simulink model "finalmodel2"  (R2024b)
settings: Solver=ode4  StartTime=0.0  StopTime=110.0  FixedStep=SampleTime  MaxStep=1e-3  RelTol=1e-4  AbsTol=1e-3
values from neighbouring files (symbols this model uses):
  Cf = 0.00911825194797    [finalmodel2.mat]    (also in finalmodel3.mat)
  D = 6191.85011148    [finalmodel2.mat]    (also in finalmodel3.mat)
  J = 773.981263935    [finalmodel2.mat]    (also in finalmodel3.mat)
  k10 = 1    [finalmodel2.mat]    (also in finalmodel3.mat)
  k11 = 25    [finalmodel2.mat]    (also in finalmodel3.mat)
  k12 = 1    [finalmodel2.mat]    (also in finalmodel3.mat)
  k13 = 120    [finalmodel2.mat]    (also in finalmodel3.mat)
  k14 = 1    [finalmodel2.mat]    (also in finalmodel3.mat)
  k2 = 9.4    [finalmodel2.mat]    (also in finalmodel3.mat)
  k3 = 1    [finalmodel2.mat]    (also in finalmodel3.mat)
  k4 = 25    [finalmodel2.mat]    (also in finalmodel3.mat)
  k5 = 1    [finalmodel2.mat]    (also in finalmodel3.mat)
  k6 = 120    [finalmodel2.mat]    (also in finalmodel3.mat)
  k7 = 1    [finalmodel2.mat]    (also in finalmodel3.mat)
  k9 = 9.4    [finalmodel2.mat]    (also in finalmodel3.mat)
  Kip_vsg = 0.00606060606061    [finalmodel2.mat]    (also in finalmodel3.mat)
  Kq_vsg = 1.48453923805e-06    [finalmodel2.mat]    (also in finalmodel3.mat)
  Kvi_vsg = 899.93539556    [finalmodel2.mat]    (also in finalmodel3.mat)
  Kvp_vsg = 5.72916666667    [finalmodel2.mat]    (also in finalmodel3.mat)
  L1 = 1.15749049521e-05    [finalmodel2.mat]    (also in finalmodel3.mat)
  Ls = 1.92915082536e-06    [finalmodel2.mat]    (also in finalmodel3.mat)
  Pset = 8281000    [finalmodel2.mat]    (also in finalmodel3.mat = 8280000)
  R1 = 0.000290909090909    [finalmodel2.mat]    (also in finalmodel3.mat)
  SampleTime = 5e-05    [finalmodel2.mat]    (also in finalmodel3.mat)
  Us = 326.598632371    [finalmodel2.mat]    (also in finalmodel3.mat)
  Vdclink = 800    [finalmodel2.mat]    (also in finalmodel3.mat)
  wn = 376.991118431    [finalmodel2.mat]    (also in finalmodel3.mat)
undefined symbols (not defined in the file or in its folder): sigbuilder_block
libraries: spsThreePhaseVIMeasurementLib x15, spsLoadFlowBusLib x9, spsThreePhasePISectionLineLib x6, spsThreePhaseTransformerTwoWindingsLib x4, spsThreePhaseParallelRLCLoadLib x4, spsabctodq0Lib x4, spsThreePhaseSeriesRLCBranchLib x3, spsSynchronousMachinepuStandardLib x2, spsExcitationSystemLib x2, spsMultiBandPowerSystemStabilizerLib x2, spsSteamTurbineandGovernorLib x2, spsGroundLib x2
(part 1 of 3)
settings Model: SimulationMode=accelerator  Creator=jp536285  LastModifiedBy=Raju
settings SolverCC: AutoScaleAbsTol=off  InitialStep=1e-5  ZeroCrossControl=DisableAll  AlgebraicLoopSolver=TrustRegion  AutoInsertRateTranBlk=on
settings DataIOCC: MaxDataPoints=100000
settings OptimizationCC: LifeSpan=inf
settings DebuggingCC: UnderspecifiedInitializationDetection=Classic  MergeDetectMultiDrivingBlocksExec=none  MultiTaskRateTransMsg=warning  IntegerOverflowMsg=none  StateNameClashWarn=warning  SFUnexpectedBacktrackingDiag=warning  SFNoUnconditionalDefaultTransitionDiag=warning  ArithmeticOperatorsInVariantConditions=warning
settings HardwareCC: ProdBitPerPointer=32  ProdBitPerSizeT=32  ProdBitPerPtrDiffT=32  ProdLargestAtomicFloat=None  ProdIntDivRoundTo=Undefined  ProdEndianess=Unspecified  ProdWordSize=32  ProdHWDeviceType=32-bit Generic
settings ModelReferenceCC: EnableRefExpFcnMdlSchedulingChecks=on  PropagateSignalLabelsOutOfModel=off
settings SFSimCC: SimUseLocalCustomCode=off  CustomCodeUndefinedFunction=UseInterfaceOnly
settings RTWCC: RTWUseLocalCustomCode=off  GPUComputeCapability=3.5
settings CodeAppCC: StateflowObjectComments=on
settings GRTTargetCC: TargetLangStandard=C89/C90 (ANSI)
settings ConfigComp: CovMetricSettings=dw  CovSaveCumulativeToWorkspaceVar=on  CovSaveSingleToWorkspaceVar=on  CovExternalEMLEnable=off
settings SimscapeCC: SimscapeNormalizeSystem=off

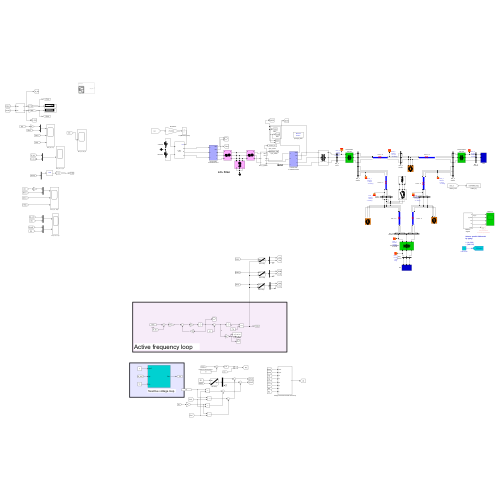
[thumbnail: Simulink's stored preview of the top-level diagram]
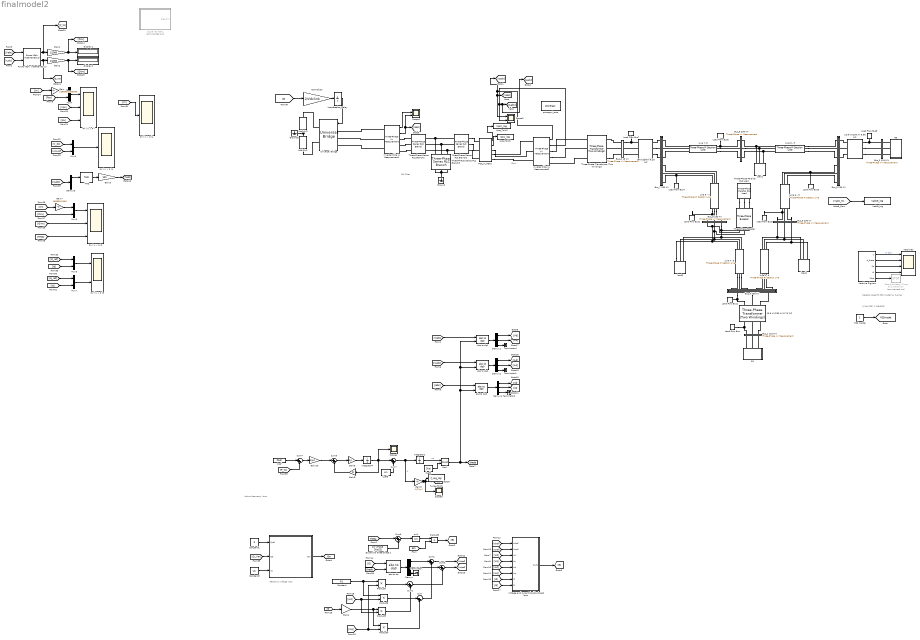
== system finalmodel2 ==
  note: Select a specific PSS model
      | by typing:
  note: 0  (No PSS)
      | 1  (MB-PSS)
  note: Grid
  note: LCL Filter
  note: Reactive voltage loop
  note: Active frequency loop
  " " : Subsystem
  " Line 4 - 6" : spsThreePhasePISectionLineLib/Three-Phase PI Section Line  LConnTagsString=a|b|c  RConnTagsString=A|B|C  Length=100  Frequency=60  Resistances=[ 0.08993 0.224825]  Inductances="[ 1.29e-3  3.22e-3]"  Capacitances="[ 9.5e-9  6.5e-9 ]"  mask(Three-Phase PI Section Line){}
      mask Display:
      | % This is a new mask on top of the base mask.
      | % Use "View base mask" link below to see the base mask.
      | patch([0.0 0.0 1 1 0.0 0.0 ],[0.4 0.7 0.7 0.4 0.4 0.7],[0 0 1]);
      | patch([0.4 0.4 0.42 0.42],[0.4 0.75 0.75 0.4],[1 0 0]);
      | patch([0.38 0.38 0.57 0.57],[0.7 0.75 0.75 0.7],[1 0 0]);
      | patch([0.53 0.53 0.55 0.55],[0.4 0.75 0.75 0.4],[1 0 0]);
  " Line 6 - 9" : spsThreePhasePISectionLineLib/Three-Phase PI Section Line  LConnTagsString=a|b|c  RConnTagsString=A|B|C  Length=100  Frequency=60  Resistances=[ 0.20631 0.5157]  Inductances="[ 2.38e-3  6.09e-3]"  Capacitances=[17.95e-9 10.55e-9]  mask(Three-Phase PI Section Line){}
      mask Display:
      | % This is a new mask on top of the base mask.
      | % Use "View base mask" link below to see the base mask.
      | patch([0.0 0.0 1 1 0.0 0.0 ],[0.4 0.7 0.7 0.4 0.4 0.7],[0 0 1]);
      | patch([0.4 0.4 0.42 0.42],[0.4 0.75 0.75 0.4],[1 0 0]);
      | patch([0.38 0.38 0.57 0.57],[0.7 0.75 0.75 0.7],[1 0 0]);
      | patch([0.53 0.53 0.55 0.55],[0.4 0.75 0.75 0.4],[1 0 0]);
  13.8 KV/230 KV 5.86 %Z : spsThreePhaseTransformerTwoWindingsLib/Three-Phase Transformer (Two Windings)  Winding1Connection=Yg  Winding2Connection=Yg  CoreType=Three single-phase transformers  SetSaturation=off  Hysteresis=off  DataFile='hysteresis'  SetInitialFlux=off  Measurements=None  UNITS=pu  NominalPower=[ 100e6 , 60 ]  Winding1=[ 13.8e3 , 1e-6 , 0 ]  Winding2=[ 230e3 , 1e-6, 0.0586 ]  Rm=500  Lm=500  L0=0.5  Saturation=[ 0,0 ; 0.0024,1.2 ; 1.0,1.52 ]  InitialFluxes=[ 0.8 , -0.8 , 0.7 ]  BreakLoop=off  DiscreteSolver=Trapezoidal iterative  DataType=off  TransfoNumber=1
  "16.5 KV/230 KV 5.76 %Z     " : spsThreePhaseTransformerTwoWindingsLib/Three-Phase Transformer (Two Windings)  Winding1Connection=Yg  Winding2Connection=Yg  CoreType=Three single-phase transformers  SetSaturation=off  Hysteresis=off  DataFile='hysteresis'  SetInitialFlux=off  Measurements=None  UNITS=pu  NominalPower=[ 100e6 , 60 ]  Winding1=[ 16.5e3 , 1e-6, 0 ]  Winding2=[ 230e3 ,1e-6, 0.0576 ]  Rm=500  Lm=500  L0=0.5  Saturation=[ 0,0 ; 0.0024,1.2 ; 1.0,1.52 ]  InitialFluxes=[ 0.8 , -0.8 , 0.7 ]  BreakLoop=off  DiscreteSolver=Trapezoidal iterative  DataType=off  TransfoNumber=1
  18KV/230KV 6.25 %Z : spsThreePhaseTransformerTwoWindingsLib/Three-Phase Transformer (Two Windings)  Winding1Connection=Yg  Winding2Connection=Yg  CoreType=Three single-phase transformers  SetSaturation=off  Hysteresis=off  DataFile='hysteresis'  SetInitialFlux=off  Measurements=None  UNITS=pu  NominalPower=[ 100e6 , 60 ]  Winding1=[ 18e3 , 1e-6 , 0]  Winding2=[ 230e3 , 1e-6, 0.0625 ]  Rm=500  Lm=500  L0=0.5  Saturation=[ 0,0 ; 0.0024,1.2 ; 1.0,1.52 ]  InitialFluxes=[ 0.8 , -0.8 , 0.7 ]  BreakLoop=off  DiscreteSolver=Trapezoidal iterative  DataType=off  TransfoNumber=1
  Bus_1 16.5 KV : spsThreePhaseVIMeasurementLib/Three-Phase V-I Measurement  VoltageMeasurement=phase-to-ground  SetLabelV=on  LabelV=Vabc_1  Vpu=on  VpuLL=off  CurrentMeasurement=yes  SetLabelI=on  LabelI=Iabc_1  Ipu=on  Pbase=100e6  Vbase=16.5e3  OutputType=Complex  PhasorSimulation=off  PSBequivalent=0
  Bus_2 18 KV : spsThreePhaseVIMeasurementLib/Three-Phase V-I Measurement  VoltageMeasurement=phase-to-ground  SetLabelV=on  LabelV=Vabc_2  Vpu=on  VpuLL=off  CurrentMeasurement=yes  SetLabelI=on  LabelI=Iabc_2  Ipu=on  Pbase=100e6  Vbase=18e3  OutputType=Complex  PhasorSimulation=off  PSBequivalent=0
  Bus_3 13.8 KV : spsThreePhaseVIMeasurementLib/Three-Phase V-I Measurement  VoltageMeasurement=phase-to-ground  SetLabelV=on  LabelV=Vabc_3  Vpu=on  VpuLL=off  CurrentMeasurement=yes  SetLabelI=on  LabelI=Iabc_3  Ipu=on  Pbase=100e6  Vbase=13.8e3  OutputType=Complex  PhasorSimulation=off  PSBequivalent=0
  Bus_4 230 KV : Subsystem
  Bus_5 230 KV : spsThreePhaseVIMeasurementLib/Three-Phase V-I Measurement  VoltageMeasurement=phase-to-ground  SetLabelV=on  LabelV=Vabc_5  Vpu=on  VpuLL=off  CurrentMeasurement=yes  SetLabelI=on  LabelI=Iabc_5  Ipu=on  Pbase=100e6  Vbase=230e3  OutputType=Complex  PhasorSimulation=off  PSBequivalent=0
  Bus_6 230 KV : spsThreePhaseVIMeasurementLib/Three-Phase V-I Measurement  VoltageMeasurement=phase-to-phase  SetLabelV=on  LabelV=Vabc_6  Vpu=off  VpuLL=on  CurrentMeasurement=yes  SetLabelI=on  LabelI=Iabc_6  Ipu=on  Pbase=100e6  Vbase=230e3  OutputType=Complex  PhasorSimulation=off  PSBequivalent=0
  Bus_7 230 KV : Subsystem
  Bus_8 230 KV : spsThreePhaseVIMeasurementLib/Three-Phase V-I Measurement  VoltageMeasurement=phase-to-phase  SetLabelV=on  LabelV=Vabc_8  Vpu=off  VpuLL=on  CurrentMeasurement=yes  SetLabelI=on  LabelI=Iabc_8  Ipu=on  Pbase=100e6  Vbase=230e3  OutputType=Complex  PhasorSimulation=off  PSBequivalent=0
  Bus_9 230 KV : Subsystem
  Constant : Constant  Value=R1
  Constant1 : Constant  Value=0
  Constant2 : Constant  Value=Us
  Demux{,1..4} (5 alike) : Demux  Outputs=3
      Demux1 settings: DisplayOption=none
      Demux2 settings: DisplayOption=none
      Demux4 settings: DisplayOption=none
  Display1 : Display
      settings: SampleTime=SampleTime
  Display2 : Display
      settings: SampleTime=SampleTime
  Expand to three-phase 1 : Constant  Value=[0 -2*pi/3 2*pi/3]
  G1 : Subsystem
  G3 : Subsystem
  Gain : Gain  Gain=108830/1000000  SampleTime=SampleTime
  Gain1 : Gain  Gain=1/1000  SampleTime=SampleTime
  Gain10 : Gain  Gain=1/wn
  Gain2 : Gain  Gain=1/1000  SampleTime=SampleTime
  Gain3 : Gain  Gain=100  SampleTime=SampleTime
  Gain4 : Gain  Gain=L1*2*pi
  Gain5 : Gain  Gain=1/J
  Gain7 : Gain  Gain=108830/1000  SampleTime=SampleTime
  Gain8 : Gain  Gain=D
  Gain9 : Gain  Gain=1/(2*pi)
  "Ground " : spsGroundLib/Ground  LConnTagsString=a
  Ground3 : spsGroundLib/Ground  LConnTagsString=a
  Integrator1 : Integrator
  Integrator4 : Integrator
  Inverter Side V-I Measurement1 : spsThreePhaseVIMeasurementLib/Three-Phase V-I Measurement  VoltageMeasurement=phase-to-phase  SetLabelV=off  LabelV=Vabc  Vpu=off  VpuLL=off  CurrentMeasurement=yes  SetLabelI=off  LabelI=Iabc  Ipu=off  Pbase=100e6  Vbase=500e3  OutputType=Complex  PhasorSimulation=off  PSBequivalent=0
  Inverter Side V-I Measurement2 : spsThreePhaseVIMeasurementLib/Three-Phase V-I Measurement  VoltageMeasurement=phase-to-ground  SetLabelV=off  LabelV=Vabc  Vpu=off  VpuLL=off  CurrentMeasurement=yes  SetLabelI=off  LabelI=Iabc  Ipu=off  Pbase=100e6  Vbase=500e3  OutputType=Complex  PhasorSimulation=off  PSBequivalent=0
  Ipcc_ToWS : ToWorkspace  VariableName=Ipcc_log  SaveFormat=Timeseries  SampleTime=SampleTime
  "Line 4 - 5 " : spsThreePhasePISectionLineLib/Three-Phase PI Section Line  LConnTagsString=a|b|c  RConnTagsString=A|B|C  Length=100  Frequency=60  Resistances=[ 0.0529 0.13225]  Inductances="[ 1.192e-3  2.38e-3]"  Capacitances="[ 9.5e-9  6.5e-9 ]"  mask(Three-Phase PI Section Line){}
      mask Display:
      | % This is a new mask on top of the base mask.
      | % Use "View base mask" link below to see the base mask.
      | patch([0.0 0.0 1 1 0.0 0.0 ],[0.4 0.7 0.7 0.4 0.4 0.7],[0 0 1]);
      | patch([0.4 0.4 0.42 0.42],[0.4 0.75 0.75 0.4],[1 0 0]);
      | patch([0.38 0.38 0.57 0.57],[0.7 0.75 0.75 0.7],[1 0 0]);
      | patch([0.53 0.53 0.55 0.55],[0.4 0.75 0.75 0.4],[1 0 0]);
  "Line 5 - 7 " : spsThreePhasePISectionLineLib/Three-Phase PI Section Line  LConnTagsString=a|b|c  RConnTagsString=A|B|C  Length=100  Frequency=60  Resistances=[ 0.16928 0.4232]  Inductances="[ 2.259e-3  5.64e-3]"  Capacitances=[15.34e-9 9.025e-9]  mask(Three-Phase PI Section Line){}
      mask Display:
      | % This is a new mask on top of the base mask.
      | % Use "View base mask" link below to see the base mask.
      | patch([0.0 0.0 1 1 0.0 0.0 ],[0.4 0.7 0.7 0.4 0.4 0.7],[0 0 1]);
      | patch([0.4 0.4 0.42 0.42],[0.4 0.75 0.75 0.4],[1 0 0]);
      | patch([0.38 0.38 0.57 0.57],[0.7 0.75 0.75 0.7],[1 0 0]);
      | patch([0.53 0.53 0.55 0.55],[0.4 0.75 0.75 0.4],[1 0 0]);
  Line 7- 8 : spsThreePhasePISectionLineLib/Three-Phase PI Section Line  LConnTagsString=a|b|c  RConnTagsString=A|B|C  Length=100  Frequency=60  Resistances=[0.044965 0.11241]  Inductances="[ 1.01e-3  2.02e-3]"  Capacitances="[ 12.5e-9  6.5e-9 ]"  mask(Three-Phase PI Section Line){}
      mask Display:
      | % This is a new mask on top of the base mask.
      | % Use "View base mask" link below to see the base mask.
      | patch([0.0 0.0 1 1 0.0 0.0 ],[0.4 0.7 0.7 0.4 0.4 0.7],[0 0 1]);
      | patch([0.4 0.4 0.42 0.42],[0.4 0.75 0.75 0.4],[1 0 0]);
      | patch([0.38 0.38 0.57 0.57],[0.7 0.75 0.75 0.7],[1 0 0]);
      | patch([0.53 0.53 0.55 0.55],[0.4 0.75 0.75 0.4],[1 0 0]);
  Line 8 - 9 : spsThreePhasePISectionLineLib/Three-Phase PI Section Line  LConnTagsString=a|b|c  RConnTagsString=A|B|C  Length=100  Frequency=60  Resistances=[ 0.062951 0.15737]  Inductances="[ 1.414e-3  3.53e-3]"  Capacitances=[10.47e-9 6.15e-9]  mask(Three-Phase PI Section Line){}
      mask Display:
      | % This is a new mask on top of the base mask.
      | % Use "View base mask" link below to see the base mask.
      | patch([0.0 0.0 1 1 0.0 0.0 ],[0.4 0.7 0.7 0.4 0.4 0.7],[0 0 1]);
      | patch([0.4 0.4 0.42 0.42],[0.4 0.75 0.75 0.4],[1 0 0]);
      | patch([0.38 0.38 0.57 0.57],[0.7 0.75 0.75 0.7],[1 0 0]);
      | patch([0.53 0.53 0.55 0.55],[0.4 0.75 0.75 0.4],[1 0 0]);
  Load Flow Bus : spsLoadFlowBusLib/Load Flow Bus  LConnTagsString=a  Phases=single  Connectors=on one side  ID=BUS_1  Vbase=16.5e3  Vref=1.04  Vangle=0  VLF=1.04  VLFb=1  VLFc=1  angleLF=0  angleLFb=0  angleLFc=0
      settings: AttributesFormatString=%<ID>\n%<Vbase>V\n%<VLF>pu\n%<angleLF>deg.
  Load Flow Bus1 : spsLoadFlowBusLib/Load Flow Bus  LConnTagsString=a  Phases=single  Connectors=on one side  ID=BUS_4  Vbase=230e3  Vref=1  Vangle=0  VLF=1.029  VLFb=1  VLFc=1  angleLF=-7.275  angleLFb=0  angleLFc=0
      settings: AttributesFormatString=%<ID>\n%<Vbase>V\n%<VLF>pu\n%<angleLF>deg.
  Load Flow Bus2 : spsLoadFlowBusLib/Load Flow Bus  LConnTagsString=a  Phases=single  Connectors=on one side  ID=BUS_5  Vbase=230e3  Vref=1  Vangle=0  VLF=1.002  VLFb=1  VLFc=1  angleLF=-13.97  angleLFb=0  angleLFc=0
      settings: AttributesFormatString=%<ID>\n%<Vbase>V\n%<VLF>pu\n%<angleLF>deg.
  Load Flow Bus3 : spsLoadFlowBusLib/Load Flow Bus  LConnTagsString=a  Phases=single  Connectors=on one side  ID=BUS_6  Vbase=230e3  Vref=1  Vangle=0  VLF=1.017  VLFb=1  VLFc=1  angleLF=-11.82  angleLFb=0  angleLFc=0
      settings: AttributesFormatString=%<ID>\n%<Vbase>V\n%<VLF>pu\n%<angleLF>deg.
  Load Flow Bus4 : spsLoadFlowBusLib/Load Flow Bus  LConnTagsString=a  Phases=single  Connectors=on one side  ID=BUS_7  Vbase=230e3  Vref=1  Vangle=0  VLF=1.025  VLFb=1  VLFc=1  angleLF=-15.86  angleLFb=0  angleLFc=0
      settings: AttributesFormatString=%<ID>\n%<Vbase>V\n%<VLF>pu\n%<angleLF>deg.
  Load Flow Bus5 : spsLoadFlowBusLib/Load Flow Bus  LConnTagsString=a  Phases=single  Connectors=on one side  ID=BUS_9  Vbase=230e3  Vref=1  Vangle=0  VLF=1.031  VLFb=1  VLFc=1  angleLF=-11.92  angleLFb=0  angleLFc=0
      settings: AttributesFormatString=%<ID>\n%<Vbase>V\n%<VLF>pu\n%<angleLF>deg.
  Load Flow Bus6 : spsLoadFlowBusLib/Load Flow Bus  LConnTagsString=a  Phases=single  Connectors=on one side  ID=BUS_8  Vbase=230e3  Vref=1  Vangle=0  VLF=1.017  VLFb=1  VLFc=1  angleLF=-16.48  angleLFb=0  angleLFc=0
      settings: AttributesFormatString=%<ID>\n%<Vbase>V\n%<VLF>pu\n%<angleLF>deg.
  Load Flow Bus7 : spsLoadFlowBusLib/Load Flow Bus  LConnTagsString=a  Phases=single  Connectors=on one side  ID=BUS_2  Vbase=18e3  Vref=1.025  Vangle=0  VLF=1.025  VLFb=1  VLFc=1  angleLF=-15.88  angleLFb=0  angleLFc=0
      settings: AttributesFormatString=%<ID>\n%<Vbase>V\n%<VLF>pu\n%<angleLF>deg.
  Load Flow Bus8 : spsLoadFlowBusLib/Load Flow Bus  LConnTagsString=a  Phases=single  Connectors=on one side  ID=BUS_3  Vbase=13.8e3  Vref=1.025  Vangle=0  VLF=1.025  VLFb=1  VLFc=1  angleLF=-9.229  angleLFb=0  angleLFc=0
      settings: AttributesFormatString=%<ID>\n%<Vbase>V\n%<VLF>pu\n%<angleLF>deg.
  LoopBreaker_Delay : UnitDelay  SampleTime=SampleTime  HasFrameUpgradeWarning=on
  Machine Signals : Subsystem
  Machines : Scope  NumInputPorts=4
  Mod : Math  Operator=mod  SignedPower=on
  Mux{3..7} (5 alike) : Mux  Inputs=2
  Normalizer : Gain  Gain=2/Vdclink
  PCC_VI_Meas : spsThreePhaseVIMeasurementLib/Three-Phase V-I Measurement  VoltageMeasurement=phase-to-ground  SetLabelV=off  LabelV=Vabc  Vpu=off  VpuLL=off  CurrentMeasurement=yes  SetLabelI=off  LabelI=Iabc  Ipu=off  Pbase=100e6  Vbase=500e3  OutputType=Complex  PhasorSimulation=off  PSBequivalent=0
  PSS model : Constant  SampleTime=SampleTime
  "PV ( V, I, P )" : Scope  NumInputPorts=3
  "PV ( V, I, P )1" : Scope
  "PV ( V, I, P )2" : Scope  NumInputPorts=3
  "PV ( V, I, P )3" : Scope  NumInputPorts=2
  "PV ( V, I, P )4" : Scope
  "Power (3ph, Instantaneous)" : spsPower3phInstantaneousLib/Power (3ph, Instantaneous)
  Pref : Constant  Value=Pset
  Product{3..7} (5 alike) : Product
  Scope1 : Scope  NumInputPorts=2
  Scope2 : Scope  NumInputPorts=2
  Scope3 : Scope
  Scope4 : Scope
  Signal Builder2 : Subsystem  Tag=STV Subsys  Commented=on  LoadFcn=sigbuilder_block('load');  StartFcn=sigbuilder_block('start');  StopFcn=sigbuilder_block('stop');  ClipboardFcn=sigbuilder_block('clipboard');  mask(Sigbuilder block){tuvar=[0:10]}
      mask help: Simulink:masks:SigbuilderBlock_MD
      mask init:
      | if ~strcmp(get_param(bdroot(gcbh),'SimulationStatus'),'stopped') tuvar = sigbuilder_block('maskInit'); end
      settings: CopyFcn=sigbuilder_block('copy');  DeleteFcn=sigbuilder_block('delete');  ModelCloseFcn=sigbuilder_block('modelClose');  PreSaveFcn=sigbuilder_block('preSave');  PauseFcn=sigbuilder_block('pause');  ContinueFcn=sigbuilder_block('continue');  NameChangeFcn=sigbuilder_block('namechange');  OpenFcn=sigbuilder_block('open',[220.2 153.6 550.8 361.2 ]);  CloseFcn=sigbuilder_block('close');
      mask Display: plot(0, 0, 100, 100,[2, 2, 32, 32, 2], [68, 8, 8, 68, 68],[32, 2], [38, 38], [32, 19, 2],[53, 60, 44], [32, 17, 17, 2],[16, 16, 31, 31]);txt = getActiveGroup(gcbh);text(2, 100, txt,'verticalAlignment', 'top');
  Stop simulation if loss of synchronism : Stop  Commented=on
  Sum : Sum  Inputs=|-+
  Sum{1..2,6..7} (4 alike) : Sum  Inputs=|++
  Sum3 : Sum  Inputs=|+-
  Sum4 : Sum  Inputs=|+-
  Sum5 : Sum  Inputs=|+-
  THD : spsTHDLib/THD  Freq=50  Ts=SampleTime
      link override In: SampleTime=SampleTime
      link override Mean: Ts=SampleTime
      link override Mean/In: SampleTime=SampleTime
      link override Mean/Mean: SampleTime=SampleTime
      link override Mean/Model/Digital  Clock: SampleTime=SampleTime
      link override Mean/Model/Discrete Variable Time Delay: Ts=SampleTime
      link override Mean/Model/Discrete Variable Time Delay/D: SampleTime=SampleTime
      link override Mean/Model/Discrete Variable Time Delay/In: SampleTime=SampleTime
      link override Mean/Model/Discrete Variable Time Delay/Out: SampleTime=SampleTime
      link override Mean/Model/Integ4: SampleTime=SampleTime
      link override Mean/Model/K1: SampleTime=SampleTime
      link override Mean/Model/K2: SampleTime=SampleTime
      link override Mean/Model/Relational Operator: SampleTime=SampleTime
      link override Mean/Model/Unit Delay: SampleTime=SampleTime
      link override Mean/Model/Unit Delay1: SampleTime=SampleTime
      link override RMS1: Ts=SampleTime
      link override RMS1/In: SampleTime=SampleTime
      link override RMS1/RMS: SampleTime=SampleTime
      link override RMS1/RMS /Fourier1: Ts=SampleTime
      link override RMS1/RMS /Fourier1/In: SampleTime=SampleTime
      link override RMS1/RMS /Fourier1/Mag: SampleTime=SampleTime
      link override RMS1/RMS /Fourier1/Mean: Ts=SampleTime
      link override RMS1/RMS /Fourier1/Mean value1: Ts=SampleTime
      link override RMS1/RMS /Fourier1/Mean value1/In: SampleTime=SampleTime
      link override RMS1/RMS /Fourier1/Mean value1/Mean: SampleTime=SampleTime
      link override RMS1/RMS /Fourier1/Mean value1/Model/Digital  Clock: SampleTime=SampleTime
      link override RMS1/RMS /Fourier1/Mean value1/Model/Discrete Variable Time Delay: Ts=SampleTime
      link override RMS1/RMS /Fourier1/Mean value1/Model/Discrete Variable Time Delay/D: SampleTime=SampleTime
      link override RMS1/RMS /Fourier1/Mean value1/Model/Discrete Variable Time Delay/In: SampleTime=SampleTime
      link override RMS1/RMS /Fourier1/Mean value1/Model/Discrete Variable Time Delay/Out: SampleTime=SampleTime
      link override RMS1/RMS /Fourier1/Mean value1/Model/Integ4: SampleTime=SampleTime
      link override RMS1/RMS /Fourier1/Mean value1/Model/K1: SampleTime=SampleTime
      link override RMS1/RMS /Fourier1/Mean value1/Model/K2: SampleTime=SampleTime
      link override RMS1/RMS /Fourier1/Mean value1/Model/Relational Operator: SampleTime=SampleTime
      link override RMS1/RMS /Fourier1/Mean value1/Model/Unit Delay: SampleTime=SampleTime
      link override RMS1/RMS /Fourier1/Mean value1/Model/Unit Delay1: SampleTime=SampleTime
      link override RMS1/RMS /Fourier1/Mean/In: SampleTime=SampleTime
      link override RMS1/RMS /Fourier1/Mean/Mean: SampleTime=SampleTime
      link override RMS1/RMS /Fourier1/Mean/Model/Digital  Clock: SampleTime=SampleTime
      link override RMS1/RMS /Fourier1/Mean/Model/Discrete Variable Time Delay: Ts=SampleTime
      link override RMS1/RMS /Fourier1/Mean/Model/Discrete Variable Time Delay/D: SampleTime=SampleTime
      link override RMS1/RMS /Fourier1/Mean/Model/Discrete Variable Time Delay/In: SampleTime=SampleTime
      link override RMS1/RMS /Fourier1/Mean/Model/Discrete Variable Time Delay/Out: SampleTime=SampleTime
      link override RMS1/RMS /Fourier1/Mean/Model/Integ4: SampleTime=SampleTime
      link override RMS1/RMS /Fourier1/Mean/Model/K1: SampleTime=SampleTime
      link override RMS1/RMS /Fourier1/Mean/Model/K2: SampleTime=SampleTime
      link override RMS1/RMS /Fourier1/Mean/Model/Relational Operator: SampleTime=SampleTime
      link override RMS1/RMS /Fourier1/Mean/Model/Unit Delay: SampleTime=SampleTime
      link override RMS1/RMS /Fourier1/Mean/Model/Unit Delay1: SampleTime=SampleTime
      link override RMS1/RMS /Fourier1/Phase: SampleTime=SampleTime
      link override RMS1/RMS /Fourier1/cos(wt): SampleTime=SampleTime
      link override RMS1/RMS /Fourier1/sin(wt): SampleTime=SampleTime
      link override RMS1/TrueRMS /Mean value: Ts=SampleTime
      link override RMS1/TrueRMS /Mean value/In: SampleTime=SampleTime
      link override RMS1/TrueRMS /Mean value/Mean: SampleTime=SampleTime
      link override RMS1/TrueRMS /Mean value/Model/Digital  Clock: SampleTime=SampleTime
      link override RMS1/TrueRMS /Mean value/Model/Discrete Variable Time Delay: Ts=SampleTime
      link override RMS1/TrueRMS /Mean value/Model/Discrete Variable Time Delay/D: SampleTime=SampleTime
      link override RMS1/TrueRMS /Mean value/Model/Discrete Variable Time Delay/In: SampleTime=SampleTime
      link override RMS1/TrueRMS /Mean value/Model/Discrete Variable Time Delay/Out: SampleTime=SampleTime
      link override RMS1/TrueRMS /Mean value/Model/Integ4: SampleTime=SampleTime
      link override RMS1/TrueRMS /Mean value/Model/K1: SampleTime=SampleTime
      link override RMS1/TrueRMS /Mean value/Model/K2: SampleTime=SampleTime
      link override RMS1/TrueRMS /Mean value/Model/Relational Operator: SampleTime=SampleTime
      link override RMS1/TrueRMS /Mean value/Model/Unit Delay: SampleTime=SampleTime
      link override RMS1/TrueRMS /Mean value/Model/Unit Delay1: SampleTime=SampleTime
      link override RMS2: Ts=SampleTime
      link override RMS2/In: SampleTime=SampleTime
      link override RMS2/RMS: SampleTime=SampleTime
      link override RMS2/RMS /Fourier1: Ts=SampleTime
      link override RMS2/RMS /Fourier1/In: SampleTime=SampleTime
      link override RMS2/RMS /Fourier1/Mag: SampleTime=SampleTime
      link override RMS2/RMS /Fourier1/Mean: Ts=SampleTime
      link override RMS2/RMS /Fourier1/Mean value1: Ts=SampleTime
      link override RMS2/RMS /Fourier1/Mean value1/In: SampleTime=SampleTime
      link override RMS2/RMS /Fourier1/Mean value1/Mean: SampleTime=SampleTime
      link override RMS2/RMS /Fourier1/Mean value1/Model/Digital  Clock: SampleTime=SampleTime
      link override RMS2/RMS /Fourier1/Mean value1/Model/Discrete Variable Time Delay: Ts=SampleTime
      link override RMS2/RMS /Fourier1/Mean value1/Model/Discrete Variable Time Delay/D: SampleTime=SampleTime
      link override RMS2/RMS /Fourier1/Mean value1/Model/Discrete Variable Time Delay/In: SampleTime=SampleTime
      link override RMS2/RMS /Fourier1/Mean value1/Model/Discrete Variable Time Delay/Out: SampleTime=SampleTime
      link override RMS2/RMS /Fourier1/Mean value1/Model/Integ4: SampleTime=SampleTime
      link override RMS2/RMS /Fourier1/Mean value1/Model/K1: SampleTime=SampleTime
      link override RMS2/RMS /Fourier1/Mean value1/Model/K2: SampleTime=SampleTime
      link override RMS2/RMS /Fourier1/Mean value1/Model/Relational Operator: SampleTime=SampleTime
      link override RMS2/RMS /Fourier1/Mean value1/Model/Unit Delay: SampleTime=SampleTime
      link override RMS2/RMS /Fourier1/Mean value1/Model/Unit Delay1: SampleTime=SampleTime
      link override RMS2/RMS /Fourier1/Mean/In: SampleTime=SampleTime
      link override RMS2/RMS /Fourier1/Mean/Mean: SampleTime=SampleTime
      link override RMS2/RMS /Fourier1/Mean/Model/Digital  Clock: SampleTime=SampleTime
      link override RMS2/RMS /Fourier1/Mean/Model/Discrete Variable Time Delay: Ts=SampleTime
      link override RMS2/RMS /Fourier1/Mean/Model/Discrete Variable Time Delay/D: SampleTime=SampleTime
      link override RMS2/RMS /Fourier1/Mean/Model/Discrete Variable Time Delay/In: SampleTime=SampleTime
      link override RMS2/RMS /Fourier1/Mean/Model/Discrete Variable Time Delay/Out: SampleTime=SampleTime
      link override RMS2/RMS /Fourier1/Mean/Model/Integ4: SampleTime=SampleTime
      link override RMS2/RMS /Fourier1/Mean/Model/K1: SampleTime=SampleTime
      link override RMS2/RMS /Fourier1/Mean/Model/K2: SampleTime=SampleTime
      link override RMS2/RMS /Fourier1/Mean/Model/Relational Operator: SampleTime=SampleTime
      link override RMS2/RMS /Fourier1/Mean/Model/Unit Delay: SampleTime=SampleTime
      link override RMS2/RMS /Fourier1/Mean/Model/Unit Delay1: SampleTime=SampleTime
      link override RMS2/RMS /Fourier1/Phase: SampleTime=SampleTime
      link override RMS2/RMS /Fourier1/cos(wt): SampleTime=SampleTime
      link override RMS2/RMS /Fourier1/sin(wt): SampleTime=SampleTime
      link override RMS2/TrueRMS /Mean value: Ts=SampleTime
      link override RMS2/TrueRMS /Mean value/In: SampleTime=SampleTime
      link override RMS2/TrueRMS /Mean value/Mean: SampleTime=SampleTime
      link override RMS2/TrueRMS /Mean value/Model/Digital  Clock: SampleTime=SampleTime
      link override RMS2/TrueRMS /Mean value/Model/Discrete Variable Time Delay: Ts=SampleTime
      link override RMS2/TrueRMS /Mean value/Model/Discrete Variable Time Delay/D: SampleTime=SampleTime
      link override RMS2/TrueRMS /Mean value/Model/Discrete Variable Time Delay/In: SampleTime=SampleTime
      link override RMS2/TrueRMS /Mean value/Model/Discrete Variable Time Delay/Out: SampleTime=SampleTime
      link override RMS2/TrueRMS /Mean value/Model/Integ4: SampleTime=SampleTime
      link override RMS2/TrueRMS /Mean value/Model/K1: SampleTime=SampleTime
      link override RMS2/TrueRMS /Mean value/Model/K2: SampleTime=SampleTime
      link override RMS2/TrueRMS /Mean value/Model/Relational Operator: SampleTime=SampleTime
      link override RMS2/TrueRMS /Mean value/Model/Unit Delay: SampleTime=SampleTime
      link override RMS2/TrueRMS /Mean value/Model/Unit Delay1: SampleTime=SampleTime
      link override THD: SampleTime=SampleTime
  Terminator{,1..2,4} (4 alike) : Terminator
  Three-Phase Parallel RLC Load : spsThreePhaseParallelRLCLoadLib/Three-Phase Parallel RLC Load  LConnTagsString=A|B|C  Configuration=Y (grounded)  NominalVoltage=230e3  Vabc=[1e3 1e3 1e3]  Vabcp=[1e3 1e3 1e3]  NominalFrequency=60  UnbalancedPower=off  ActivePower=30000000  InductivePower=0  CapacitivePower=0  Pabc=[10e3 9e3 11e3]  QLabc=[100 90 110]  QCabc=[100 90 110]  Pabcp=[10e3 9e3 11e3]  QLabcp=[100 90 110]  QCabcp=[100 90 110]  Measurements=None  LoadType=constant Z
  Three-Phase Series RLC Branch1 : spsThreePhaseSeriesRLCBranchLib/Three-Phase Series RLC Branch  LConnTagsString=A|B|C  RConnTagsString=A|B|C  BranchType=RL  Resistance=2.9091e-05  Inductance=1.9292e-06  Capacitance=1e-6  Measurements=None
  Three-Phase Series RLC Branch2 : spsThreePhaseSeriesRLCBranchLib/Three-Phase Series RLC Branch  LConnTagsString=A|B|C  RConnTagsString=A|B|C  BranchType=RL  Resistance=2.9091e-05  Inductance=1.1575e-06  Capacitance=1e-6  Measurements=None
  Three-Phase Series RLC Branch3 : spsThreePhaseSeriesRLCBranchLib/Three-Phase Series RLC Branch  LConnTagsString=A|B|C  RConnTagsString=A|B|C  BranchType=RC  Resistance=0.0029691  Inductance=500e-6  Capacitance=0.0091183  Measurements=None
  Three-Phase Transformer (Two Windings) : spsThreePhaseTransformerTwoWindingsLib/Three-Phase Transformer (Two Windings)  Winding1Connection=Yg  Winding2Connection=Yg  CoreType=Three single-phase transformers  SetSaturation=off  Hysteresis=off  DataFile='hysteresis'  SetInitialFlux=off  Measurements=None  UNITS=pu  NominalPower=[ 200e6 , 60 ]  Winding1=[ 400 , 0.002 , 0.08 ]  Winding2=[ 18e3 , 0.002 , 0.08 ]  Rm=500  Lm=500  L0=0.5  Saturation=[ 0,0 ; 0.0024,1.2 ; 1.0,1.52 ]  InitialFluxes=[ 0.8 , -0.8 , 0.7 ]  BreakLoop=off  DiscreteSolver=Trapezoidal iterative  DataType=off  TransfoNumber=1
  Three-Phase Breaker : spsThreePhaseBreakerLib/Three-Phase Breaker  InitialState=open  SwitchA=on  SwitchB=on  SwitchC=on  SwitchTimes=[50]  External=off  BreakerResistance=0.01  SnubberResistance=1e6  SnubberCapacitance=inf  Measurements=None
      link override Breaker A/Model/C4: SampleTime=SampleTime
      link override Breaker A/Model/Timer: Ts=SampleTime
      link override Breaker A/Model/Timer/Digital Clock: SampleTime=SampleTime
      link override Breaker A/Model/Uswitch: SampleTime=SampleTime
      link override Breaker A/Model/gate: SampleTime=SampleTime
      link override Breaker B/Model/C4: SampleTime=SampleTime
      link override Breaker B/Model/Timer: Ts=SampleTime
      link override Breaker B/Model/Timer/Digital Clock: SampleTime=SampleTime
      link override Breaker B/Model/Uswitch: SampleTime=SampleTime
      link override Breaker B/Model/gate: SampleTime=SampleTime
      link override Breaker C/Model/C4: SampleTime=SampleTime
      link override Breaker C/Model/Timer: Ts=SampleTime
      link override Breaker C/Model/Timer/Digital Clock: SampleTime=SampleTime
      link override Breaker C/Model/Uswitch: SampleTime=SampleTime
      link override Breaker C/Model/gate: SampleTime=SampleTime
      link override Stair Generator: Ts=SampleTime
      link override Stair Generator/Model/Digital Clock: SampleTime=SampleTime
      link override Stair Generator/Model/Look-Up Table: SampleTime=SampleTime
      link override Stair Generator/Out: SampleTime=SampleTime
  Universal Bridge : spsUniversalBridgeLib/Universal Bridge  Arms=3  SnubberResistance=inf  SnubberCapacitance=inf  Device=Average-model based VSC  Ron=1e-3  Lon=0  ForwardVoltages="[  0  0  ]"  ForwardVoltage=0  GTOparameters=[ 10e-6 , 20e-6 ]  IGBTparameters=[ 1e-6 , 2e-6 ]  Measurements=None  Measurements_2=None  converterType=Rectifier
  Vabc5_log : ToWorkspace  VariableName=Vabc5_log  SaveFormat=Timeseries  SampleTime=-1
  Vdclink/2 : spsDCVoltageSourceLib/DC Voltage Source  Amplitude=Vdclink/2  Measurements=None
  Vdclink/2. : spsDCVoltageSourceLib/DC Voltage Source  Amplitude=Vdclink/2  Measurements=None
  Voltage and current double closed loop : Subsystem
  Vpcc_ToWS : ToWorkspace  VariableName=Vpcc_log  SaveFormat=Timeseries  SampleTime=SampleTime
  abc to dq{,1..3} (4 alike) : spsabctodq0Lib/abc to dq0  Alignment=90 degrees behind phase A axis
  f_ref1 : Constant  Value=2*pi
  f_ref5 : Constant  Value=wn
  f_vsg_ToWS : ToWorkspace  VariableName=f_vsg_log  SaveFormat=Timeseries  SampleTime=-1
  load1 : spsThreePhaseParallelRLCLoadLib/Three-Phase Parallel RLC Load  LConnTagsString=A|B|C  Configuration=Y (grounded)  NominalVoltage=(230000)*1.0168  Vabc=[1e3 1e3 1e3]  Vabcp=[1e3 1e3 1e3]  NominalFrequency=60  UnbalancedPower=off  ActivePower=100000000  InductivePower=35000000  CapacitivePower=0  Pabc=[10e3 9e3 11e3]  QLabc=[100 90 110]  QCabc=[100 90 110]  Pabcp=[10e3 9e3 11e3]  QLabcp=[100 90 110]  QCabcp=[100 90 110]  Measurements=None  LoadType=constant PQ
  load2 : spsThreePhaseParallelRLCLoadLib/Three-Phase Parallel RLC Load  LConnTagsString=A|B|C  Configuration=Y (grounded)  NominalVoltage=(230000)*1.00166  Vabc=[1e3 1e3 1e3]  Vabcp=[1e3 1e3 1e3]  NominalFrequency=60  UnbalancedPower=off  ActivePower=125000000  InductivePower=50000000  CapacitivePower=0  Pabc=[10e3 9e3 11e3]  QLabc=[100 90 110]  QCabc=[100 90 110]  Pabcp=[10e3 9e3 11e3]  QLabcp=[100 90 110]  QCabcp=[100 90 110]  Measurements=None  LoadType=constant PQ
  load4 : spsThreePhaseParallelRLCLoadLib/Three-Phase Parallel RLC Load  LConnTagsString=A|B|C  Configuration=Y (grounded)  NominalVoltage=(230000)*1.01715  Vabc=[1e3 1e3 1e3]  Vabcp=[1e3 1e3 1e3]  NominalFrequency=60  UnbalancedPower=off  ActivePower=90000000  InductivePower=30000000  CapacitivePower=0  Pabc=[10e3 9e3 11e3]  QLabc=[100 90 110]  QCabc=[100 90 110]  Pabcp=[10e3 9e3 11e3]  QLabcp=[100 90 110]  QCabcp=[100 90 110]  Measurements=None  LoadType=constant PQ
  powergui_auto : spspowerguiLib/powergui  Priority=1  SimulationMode=Discrete  SampleTime=SampleTime  frequency=60  Iterations=50  frequencyindice=60  Pbase=100e6  ErrMax=1e-4  UnitsV=kV  UnitsW=MW  buscounter=0  FunctionMessages=off  echomessages=off  EnableUseOfTLC=off  CurrentSourceSwitches=off  DisableSnubberDevices=off  DisableRonSwitches=off  DisableVfSwitches=off  DisplayEquations=off  AutomaticDiscreteSolvers=off  SolverType=Tustin/Backward Euler (TBE)  Interpol=off  ExternalGateDelay=off  methode=off  Ts=SampleTime  x0status=blocks  SPID=on  SwTol=0  HookPort=off  NonlinearTolerance=1e-4  nMaxIteration=100  ContinueOnMaxIteration=off  RestoreLinks=warning  ResistiveCurrentMeasurement=off  Frange=[0:2:500]  Ylog=off  Xlog=on  ShowGrid=off  save=off  variable=ZData  structure=0  ZoomFFT=off  StartTime=0.0  cycles=1  DisplayStyle=1  fundamental=60  FreqAxis=off  MaxFrequency=1000  frequencyindicesteady=1  RmsSteady=1  display=off
  sin1 : Trigonometry
  tag scope: Em=global, PSSmodel=global, theda=global
  wires:
  Machine Signals/1(w) -> Machines/1  "w (pu)"
  Machine Signals/2(d_theta) -> Machines/2
  Machine Signals/3(Pa) -> Machines/3
  Machine Signals/4(Vt) -> Machines/4
  PSS model/1 -> [PSSmodel]
  Machine Signals/5(Stop) -> Stop simulation if loss of synchronism/1
  "Power (3ph, Instantaneous)"/1 -> [P_W], Gain1/1
  Gain2/1 -> [Qinv], Display2/1
  [Irr] -> Gain7/1
  [Vabc] -> "Power (3ph, Instantaneous)"/1
  Inverter Side V-I Measurement2/1 -> [Vgabc], Scope2/1, [Vabc]
  [Ipv] -> "PV ( V, I, P )"/3
  [Pinv] -> Mux5/2
  Gain1/1 -> [Pinv], Display1/1
  [ILabc] -> Demux3/1
  [Irr] -> "PV ( V, I, P )4"/1
  [Qinv] -> "PV ( V, I, P )2"/2
  Mux3/1 -> "PV ( V, I, P )1"/1
  [Id] -> Mux6/2
  Gain/1 -> Mux4/1
  [Id_ref] -> Mux6/1
  Inverter Side V-I Measurement1/2 -> [Iabc], Scope1/2
  Mux5/1 -> "PV ( V, I, P )2"/1
  [V_dc] -> Mux3/1
  [Vpv] -> "PV ( V, I, P )"/2
  Inverter Side V-I Measurement1/1 -> Scope1/1
  THD/1 -> Gain3/1
  "Power (3ph, Instantaneous)"/2 -> [Q_Var], Gain2/1
  Gain3/1 -> [THDi]
  Demux3/1 -> THD/1
  Gain7/1 -> Mux5/1
  Inverter Side V-I Measurement2/2 -> Scope2/2, [Igabc], [ILabc]
  [Iq] -> Mux7/2
  [Iq_ref] -> Mux7/1
  Mux6/1 -> "PV ( V, I, P )3"/1
  [Ppv] -> Mux4/2
  [THDi] -> "PV ( V, I, P )2"/3
  [ILabc] -> "Power (3ph, Instantaneous)"/2
  Mux4/1 -> "PV ( V, I, P )"/1
  Mux7/1 -> "PV ( V, I, P )3"/2
  [V_dc_ref] -> Mux3/2
  [Irr] -> Gain/1
  [Vabc_5] -> Vabc5_log/1
  PCC_VI_Meas/1 -> Vpcc_ToWS/1
  PCC_VI_Meas/2 -> Ipcc_ToWS/1
  [Id] -> Voltage and current double closed loop/7(Id)
  Sum1/1 -> Sum3/2
  [Vq] -> Voltage and current double closed loop/4(Vq)
  [Vqref] -> Voltage and current double closed loop/2(Vqref)
  Product5/1 -> Sum1/2
  abc to dq/1 -> Demux/1
  Product7/1 -> Sum1/1
  [ILq] -> Product4/2, Product7/2
  [ILq] -> Voltage and current double closed loop/6(ILq)
  Demux/1 -> Sum2/1
  Gain4/1 -> Product4/1, Product5/1
  Product4/1 -> Sum/2
  Demux/2 -> Sum3/1
  Expand to three-phase 1/1 -> Sum6/2
  " "/1(Em) -> [Em]
  [ILd] -> Voltage and current double closed loop/5(ILd)
  [Vdref] -> Voltage and current double closed loop/1(Vdref)
  Sum/1 -> Sum2/2
  Product6/1 -> Sum/1
  [Vd] -> Voltage and current double closed loop/3(Vd)
  [theda] -> abc to dq/2
  [Iq] -> Voltage and current double closed loop/8(Iq)
  Constant1/1 -> " "/1(Qref)
  Voltage and current double closed loop/1(Out1) -> [e]
  [f] -> Gain4/1
  Constant/1 -> Product6/1, Product7/1
  [Em] -> Product3/2
  [Q_Var] -> " "/2(Qe)
  [theda] -> Sum6/1
  Sum6/1 -> sin1/1
  sin1/1 -> Product3/1
  Sum2/1 -> [Vdref]
  Constant2/1 -> " "/3(Us)
  Sum3/1 -> [Vqref]
  Demux/3 -> Terminator/1
  [E] -> abc to dq/1
  Product3/1 -> [E]
  [ILd] -> Product5/2, Product6/2
  abc to dq2/1 -> Demux2/1
  Demux1/1 -> [Vd]
  Demux1/2 -> [Vq]
  Demux4/2 -> [Iq]
  abc to dq3/1 -> Demux4/1
  Demux2/3 -> Terminator1/1
  [P_W] -> Sum4/2
  Gain8/1 -> Sum5/2
  Sum7/1 -> Integrator1/1, Gain9/1  "w"
  Demux1/3 -> Terminator4/1
  Gain9/1 -> Scope3/1, [f], f_vsg_ToWS/1
  Integrator1/1 -> Mod/1  "wt"
  [ILabc] -> abc to dq2/1
  Sum5/1 -> Gain5/1
  f_ref1/1 -> Mod/2
  Integrator4/1 -> Scope4/1, Sum7/1, Gain8/1
  abc to dq1/1 -> Demux1/1
  Demux4/3 -> Terminator2/1
  Pref/1 -> Sum4/1
  Mod/1 -> [theda], abc to dq3/2, abc to dq2/2, abc to dq1/2
  Demux2/1 -> [ILd]
  f_ref5/1 -> Sum7/2
  Gain10/1 -> Sum5/1
  [Vabc] -> abc to dq1/1
  Demux4/1 -> [Id]
  [Iabc] -> abc to dq3/1
  Gain5/1 -> Integrator4/1
  Demux2/2 -> [ILq]
  Sum4/1 -> Gain10/1
  [e] -> Normalizer/1
  Normalizer/1 -> LoopBreaker_Delay/1
  LoopBreaker_Delay/1 -> Universal Bridge/1
  connections:
  Bus_2 18 KV/LConn2 -- Three-Phase Transformer (Two Windings)/RConn2
  18KV/230KV 6.25 %Z/LConn2 -- Bus_2 18 KV/RConn2
  18KV/230KV 6.25 %Z/RConn2 -- Bus_7 230 KV/LConn2
  Bus_2 18 KV/RConn1 -- Load Flow Bus7/LConn1 -- 18KV/230KV 6.25 %Z/LConn1
  Bus_2 18 KV/RConn3 -- 18KV/230KV 6.25 %Z/LConn3
  Bus_7 230 KV/LConn1 -- 18KV/230KV 6.25 %Z/RConn1
  18KV/230KV 6.25 %Z/RConn3 -- Bus_7 230 KV/LConn3
  Load Flow Bus8/LConn1 -- 13.8 KV/230 KV 5.86 %Z/LConn1 -- Bus_3 13.8 KV/LConn1
  13.8 KV/230 KV 5.86 %Z/LConn2 -- Bus_3 13.8 KV/LConn2
  13.8 KV/230 KV 5.86 %Z/LConn3 -- Bus_3 13.8 KV/LConn3
  Bus_1 16.5 KV/LConn1 -- Load Flow Bus/LConn1 -- "16.5 KV/230 KV 5.76 %Z     "/LConn1
  Bus_1 16.5 KV/LConn3 -- "16.5 KV/230 KV 5.76 %Z     "/LConn3
  Bus_1 16.5 KV/LConn2 -- "16.5 KV/230 KV 5.76 %Z     "/LConn2
  13.8 KV/230 KV 5.86 %Z/RConn1 -- Bus_9 230 KV/RConn1
  13.8 KV/230 KV 5.86 %Z/RConn2 -- Bus_9 230 KV/RConn2
  13.8 KV/230 KV 5.86 %Z/RConn3 -- Bus_9 230 KV/RConn3
  Bus_4 230 KV/LConn1 -- Load Flow Bus1/LConn1 -- "16.5 KV/230 KV 5.76 %Z     "/RConn1
  Bus_4 230 KV/LConn2 -- "16.5 KV/230 KV 5.76 %Z     "/RConn2
  Line 8 - 9/LConn1 -- load1/LConn1 -- Bus_8 230 KV/LConn1
  Bus_8 230 KV/LConn2 -- load1/LConn2 -- Line 8 - 9/LConn2
  Line 8 - 9/LConn3 -- load1/LConn3 -- Bus_8 230 KV/LConn3
  "16.5 KV/230 KV 5.76 %Z     "/RConn3 -- Bus_4 230 KV/LConn3
  "Line 4 - 5 "/LConn3 -- Three-Phase Breaker/LConn3 -- Bus_5 230 KV/RConn3 -- load2/LConn3
  " Line 4 - 6"/LConn1 -- load4/LConn1 -- Bus_6 230 KV/RConn1
  " Line 4 - 6"/LConn2 -- load4/LConn2 -- Bus_6 230 KV/RConn2
  " Line 4 - 6"/LConn3 -- load4/LConn3 -- Bus_6 230 KV/RConn3
  Line 7- 8/LConn1 -- Bus_7 230 KV/RConn1
  Line 7- 8/LConn2 -- Bus_7 230 KV/RConn2
  Bus_7 230 KV/RConn3 -- Line 7- 8/LConn3
  Bus_8 230 KV/RConn1 -- Load Flow Bus6/LConn1 -- Line 7- 8/RConn1
  Line 7- 8/RConn2 -- Bus_8 230 KV/RConn2
  Line 7- 8/RConn3 -- Bus_8 230 KV/RConn3
  Line 8 - 9/RConn2 -- Bus_9 230 KV/LConn2
  Line 8 - 9/RConn1 -- Bus_9 230 KV/LConn1
  Line 8 - 9/RConn3 -- Bus_9 230 KV/LConn3
  "Line 5 - 7 "/RConn1 -- Load Flow Bus2/LConn1 -- Bus_5 230 KV/LConn1
  "Line 5 - 7 "/RConn2 -- Bus_5 230 KV/LConn2
  "Line 5 - 7 "/RConn3 -- Bus_5 230 KV/LConn3
  "Line 5 - 7 "/LConn1 -- Load Flow Bus4/LConn1 -- Bus_7 230 KV/RConn6
  "Line 5 - 7 "/LConn2 -- Bus_7 230 KV/RConn5
  "Line 5 - 7 "/LConn3 -- Bus_7 230 KV/RConn4
  " Line 6 - 9"/RConn1 -- Load Flow Bus5/LConn1 -- Bus_9 230 KV/LConn4
  Bus_9 230 KV/LConn5 -- " Line 6 - 9"/RConn2
  Bus_6 230 KV/LConn1 -- Load Flow Bus3/LConn1 -- " Line 6 - 9"/LConn1
  Bus_6 230 KV/LConn2 -- " Line 6 - 9"/LConn2
  Bus_6 230 KV/LConn3 -- " Line 6 - 9"/LConn3
  " Line 6 - 9"/RConn3 -- Bus_9 230 KV/LConn6
  "Line 4 - 5 "/RConn2 -- Bus_4 230 KV/RConn2
  "Line 4 - 5 "/RConn1 -- Bus_4 230 KV/RConn1
  "Line 4 - 5 "/RConn3 -- Bus_4 230 KV/RConn3
  " Line 4 - 6"/RConn2 -- Bus_4 230 KV/RConn5
  " Line 4 - 6"/RConn1 -- Bus_4 230 KV/RConn4
  " Line 4 - 6"/RConn3 -- Bus_4 230 KV/RConn6
  G3/LConn1 -- Bus_3 13.8 KV/RConn1
  G3/LConn2 -- Bus_3 13.8 KV/RConn2
  G3/LConn3 -- Bus_3 13.8 KV/RConn3
  Three-Phase Transformer (Two Windings)/RConn3 -- Bus_2 18 KV/LConn3
  Bus_2 18 KV/LConn1 -- Three-Phase Transformer (Two Windings)/RConn1
  G1/LConn1 -- Bus_1 16.5 KV/RConn1
  G1/LConn2 -- Bus_1 16.5 KV/RConn2
  G1/LConn3 -- Bus_1 16.5 KV/RConn3
  Three-Phase Series RLC Branch1/RConn2 -- Three-Phase Series RLC Branch2/LConn2 -- Three-Phase Series RLC Branch3/LConn2
  Three-Phase Series RLC Branch1/RConn3 -- Three-Phase Series RLC Branch2/LConn3 -- Three-Phase Series RLC Branch3/LConn3
  Three-Phase Series RLC Branch1/RConn1 -- Three-Phase Series RLC Branch2/LConn1 -- Three-Phase Series RLC Branch3/LConn1
  Three-Phase Series RLC Branch3/RConn1 -- Three-Phase Series RLC Branch3/RConn2 -- Three-Phase Series RLC Branch3/RConn3 -- "Ground "/LConn1
  Three-Phase Transformer (Two Windings)/LConn3 -- Inverter Side V-I Measurement2/RConn3
  Three-Phase Series RLC Branch1/LConn3 -- Inverter Side V-I Measurement1/RConn3
  Three-Phase Series RLC Branch1/LConn2 -- Inverter Side V-I Measurement1/RConn2
  Inverter Side V-I Measurement2/RConn1 -- Three-Phase Transformer (Two Windings)/LConn1
  Inverter Side V-I Measurement2/RConn2 -- Three-Phase Transformer (Two Windings)/LConn2
  Three-Phase Series RLC Branch1/LConn1 -- Inverter Side V-I Measurement1/RConn1
  Three-Phase Parallel RLC Load/LConn1 -- Three-Phase Breaker/RConn1
  Three-Phase Parallel RLC Load/LConn2 -- Three-Phase Breaker/RConn2
  Three-Phase Parallel RLC Load/LConn3 -- Three-Phase Breaker/RConn3
  load2/LConn1 -- "Line 4 - 5 "/LConn1 -- Three-Phase Breaker/LConn1 -- Bus_5 230 KV/RConn1
  load2/LConn2 -- "Line 4 - 5 "/LConn2 -- Three-Phase Breaker/LConn2 -- Bus_5 230 KV/RConn2
  Three-Phase Series RLC Branch2/RConn1 -- PCC_VI_Meas/LConn1
  PCC_VI_Meas/RConn1 -- Inverter Side V-I Measurement2/LConn1
  Three-Phase Series RLC Branch2/RConn2 -- PCC_VI_Meas/LConn2
  PCC_VI_Meas/RConn2 -- Inverter Side V-I Measurement2/LConn2
  Three-Phase Series RLC Branch2/RConn3 -- PCC_VI_Meas/LConn3
  PCC_VI_Meas/RConn3 -- Inverter Side V-I Measurement2/LConn3
  Ground3/LConn1 -- Vdclink/2/LConn1 -- Vdclink/2./RConn1
  Vdclink/2./LConn1 -- Universal Bridge/RConn2
  Inverter Side V-I Measurement1/LConn3 -- Universal Bridge/LConn3
  Inverter Side V-I Measurement1/LConn2 -- Universal Bridge/LConn2
  Inverter Side V-I Measurement1/LConn1 -- Universal Bridge/LConn1
  Universal Bridge/RConn1 -- Vdclink/2/RConn1

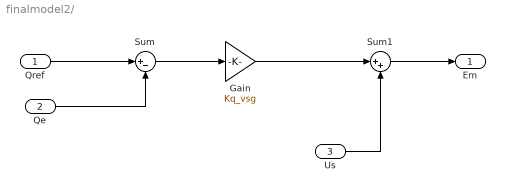
== system finalmodel2/  ==
  Qref : Inport
  Qe : Inport  Port=2
  Us : Inport  Port=3
  Gain : Gain  Gain=Kq_vsg
  Sum : Sum  Inputs=|+-
  Sum1 : Sum  Inputs=|++
  Em : Outport
  wires:
  Qref/1 -> Sum/1
  Qe/1 -> Sum/2
  Sum1/1 -> Em/1
  Us/1 -> Sum1/2
  Sum/1 -> Gain/1
  Gain/1 -> Sum1/1

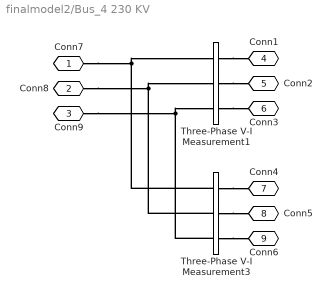
== system finalmodel2/Bus_4 230 KV ==
  Three-Phase V-I Measurement1 : spsThreePhaseVIMeasurementLib/Three-Phase V-I Measurement  VoltageMeasurement=phase-to-ground  SetLabelV=on  LabelV=Vabc_45  Vpu=on  VpuLL=off  CurrentMeasurement=yes  SetLabelI=on  LabelI=Iabc_45  Ipu=on  Pbase=100e6  Vbase=230e3  OutputType=Complex  PhasorSimulation=off  PSBequivalent=0
  Three-Phase V-I Measurement3 : spsThreePhaseVIMeasurementLib/Three-Phase V-I Measurement  VoltageMeasurement=phase-to-ground  SetLabelV=on  LabelV=Vabc_46  Vpu=on  VpuLL=off  CurrentMeasurement=yes  SetLabelI=on  LabelI=Iabc_46  Ipu=on  Pbase=100e6  Vbase=230e3  OutputType=Complex  PhasorSimulation=off  PSBequivalent=0
  Conn7 : PMIOPort  Side=Left  SampleTime=SampleTime
  Conn8 : PMIOPort  Port=2  Side=Left  SampleTime=SampleTime
  Conn9 : PMIOPort  Port=3  Side=Left  SampleTime=SampleTime
  Conn1 : PMIOPort  Port=4  Side=Right  SampleTime=SampleTime
  Conn2 : PMIOPort  Port=5  Side=Right  SampleTime=SampleTime
  Conn3 : PMIOPort  Port=6  Side=Right  SampleTime=SampleTime
  Conn4 : PMIOPort  Port=7  Side=Right  SampleTime=SampleTime
  Conn5 : PMIOPort  Port=8  Side=Right  SampleTime=SampleTime
  Conn6 : PMIOPort  Port=9  Side=Right  SampleTime=SampleTime
  connections:
  Three-Phase V-I Measurement3/LConn3 -- Conn9/RConn1 -- Three-Phase V-I Measurement1/LConn3
  Three-Phase V-I Measurement3/LConn2 -- Conn8/RConn1 -- Three-Phase V-I Measurement1/LConn2
  Three-Phase V-I Measurement3/LConn1 -- Conn7/RConn1 -- Three-Phase V-I Measurement1/LConn1
  Three-Phase V-I Measurement3/RConn3 -- Conn6/RConn1
  Three-Phase V-I Measurement1/RConn3 -- Conn3/RConn1
  Three-Phase V-I Measurement1/RConn1 -- Conn1/RConn1
  Three-Phase V-I Measurement1/RConn2 -- Conn2/RConn1
  Three-Phase V-I Measurement3/RConn1 -- Conn4/RConn1
  Three-Phase V-I Measurement3/RConn2 -- Conn5/RConn1

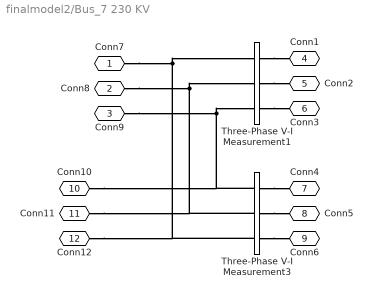
== system finalmodel2/Bus_7 230 KV ==
  Three-Phase V-I Measurement1 : spsThreePhaseVIMeasurementLib/Three-Phase V-I Measurement  VoltageMeasurement=phase-to-ground  SetLabelV=on  LabelV=Vabc_7  Vpu=on  VpuLL=off  CurrentMeasurement=yes  SetLabelI=on  LabelI=Iabc_7  Ipu=on  Pbase=100e6  Vbase=230e3  OutputType=Complex  PhasorSimulation=off  PSBequivalent=0
  Three-Phase V-I Measurement3 : spsThreePhaseVIMeasurementLib/Three-Phase V-I Measurement  VoltageMeasurement=phase-to-ground  SetLabelV=on  LabelV=Vab  Vpu=on  VpuLL=off  CurrentMeasurement=yes  SetLabelI=on  LabelI=Iab  Ipu=on  Pbase=100e6  Vbase=230e3  OutputType=Complex  PhasorSimulation=off  PSBequivalent=0
  Conn7 : PMIOPort  Side=Left  SampleTime=SampleTime
  Conn8 : PMIOPort  Port=2  Side=Left  SampleTime=SampleTime
  Conn9 : PMIOPort  Port=3  Side=Left  SampleTime=SampleTime
  Conn1 : PMIOPort  Port=4  Side=Right  SampleTime=SampleTime
  Conn2 : PMIOPort  Port=5  Side=Right  SampleTime=SampleTime
  Conn3 : PMIOPort  Port=6  Side=Right  SampleTime=SampleTime
  Conn4 : PMIOPort  Port=7  Side=Right  SampleTime=SampleTime
  Conn5 : PMIOPort  Port=8  Side=Right  SampleTime=SampleTime
  Conn6 : PMIOPort  Port=9  Side=Right  SampleTime=SampleTime
  Conn10 : PMIOPort  Port=10  Side=Left  SampleTime=SampleTime
  Conn11 : PMIOPort  Port=11  Side=Left  SampleTime=SampleTime
  Conn12 : PMIOPort  Port=12  Side=Left  SampleTime=SampleTime
  connections:
  Three-Phase V-I Measurement3/RConn2 -- Conn5/RConn1
  Three-Phase V-I Measurement3/RConn1 -- Conn4/RConn1
  Three-Phase V-I Measurement1/RConn2 -- Conn2/RConn1
  Three-Phase V-I Measurement1/RConn1 -- Conn1/RConn1
  Three-Phase V-I Measurement1/RConn3 -- Conn3/RConn1
  Three-Phase V-I Measurement3/RConn3 -- Conn6/RConn1
  Conn7/RConn1 -- Three-Phase V-I Measurement3/LConn3 -- Conn12/RConn1 -- Three-Phase V-I Measurement1/LConn1
  Conn8/RConn1 -- Three-Phase V-I Measurement3/LConn2 -- Conn11/RConn1 -- Three-Phase V-I Measurement1/LConn2
  Conn9/RConn1 -- Conn10/RConn1 -- Three-Phase V-I Measurement3/LConn1 -- Three-Phase V-I Measurement1/LConn3
